simulink model "testfrage_system"  (R2025b)
settings: Solver=ode45  StartTime=0.0  StopTime=10  MaxStep=1e-3  RelTol=1e-6  AbsTol=1e-7
settings Model: Creator=grund  LastModifiedBy=grund

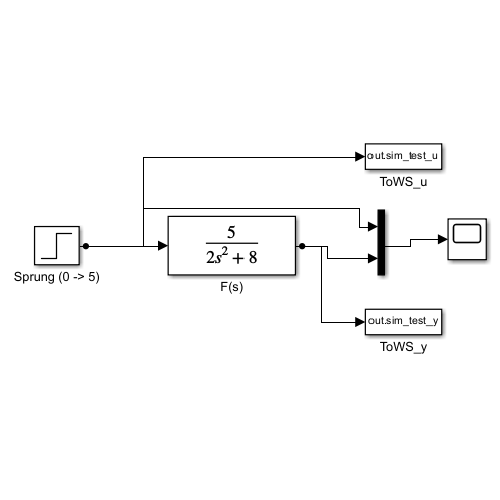
[thumbnail: Simulink's stored preview of the top-level diagram]
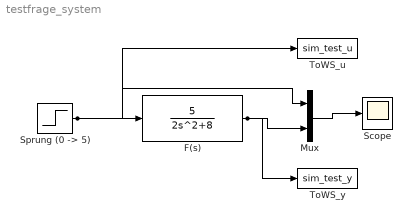
== system testfrage_system ==
  F(s) : TransferFcn  Numerator=[5]  Denominator=[2 0 8]
  Mux : Mux  Inputs=2
  Scope : Scope
  "Sprung (0 -> 5)" : Step  After=5  SampleTime=0
  ToWS_u : ToWorkspace  VariableName=sim_test_u  SaveFormat=Timeseries  SampleTime=-1
  ToWS_y : ToWorkspace  VariableName=sim_test_y  SaveFormat=Timeseries  SampleTime=-1
  wires:
  "Sprung (0 -> 5)"/1 -> F(s)/1, Mux/1, ToWS_u/1
  F(s)/1 -> Mux/2, ToWS_y/1
  Mux/1 -> Scope/1
